simulink library "dab_single_phase_pwm_modulator"  (R2025b)
settings: Solver=VariableStepAuto  StartTime=0.0  StopTime=10.0  RelTol=1e-3
settings Model: Creator=dbagn  LastModifiedBy=ltnbda

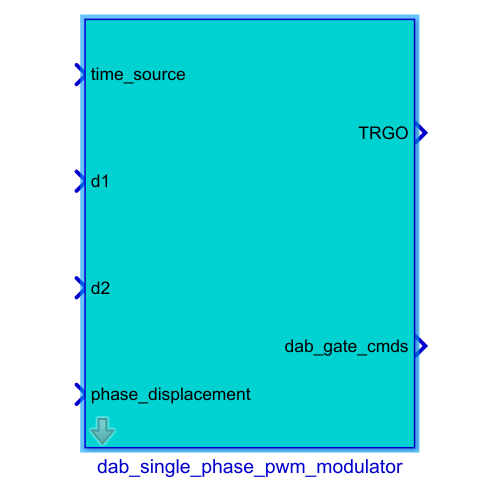
[thumbnail: Simulink's stored preview of the top-level diagram]
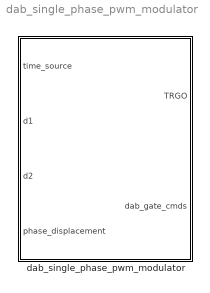
== system dab_single_phase_pwm_modulator ==
  dab_single_phase_pwm_modulator : Subsystem  mask{fPWM_DAB=10000, m_up=1, m_low=0, dead_time_DAB=0, pos_cmd_gate=18, neg_cmd_gate=-3, polarity=-1, tc=1e-6, max_phase_displacement=pi/4, trgo_double_update=0}
      mask prompts: fPWM_DAB "PWM Frequency (Hz)"; m_up "Max Input Modulation Value"; m_low "Min Input Modulation Value"; dead_time_DAB "Dead Time (s)"; pos_cmd_gate "Positive Gate Voltage cmd (V)"; neg_cmd_gate "Negative Gate Voltage cmd (V)"; polarity "Polarity (pu)"; tc "Sampling time"; max_phase_displacement "Max Phase Displacement"; trgo_double_update "TRGO double update"

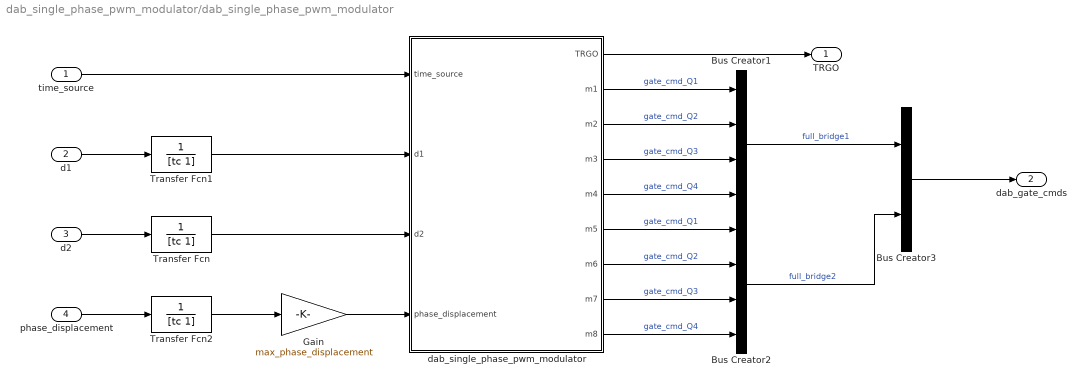
== system dab_single_phase_pwm_modulator/dab_single_phase_pwm_modulator ==
  time_source : Inport
  d1 : Inport  Port=2
  d2 : Inport  Port=3
  phase_displacement : Inport  Port=4
  Bus Creator1 : BusCreator  Inputs=4
  Bus Creator2 : BusCreator  Inputs=4
  Bus Creator3 : BusCreator  Inputs=2
  Gain : Gain  Gain=max_phase_displacement  OutDataTypeStr=double
  Transfer Fcn : TransferFcn  Denominator=[tc 1]
  Transfer Fcn1 : TransferFcn  Denominator=[tc 1]
  Transfer Fcn2 : TransferFcn  Denominator=[tc 1]
  dab_single_phase_pwm_modulator : Subsystem  mask{f=fPWM_DAB, m_up=m_up, m_low=m_low, dead_time=dead_time_DAB, pos_cmd_gate=pos_cmd_gate, neg_cmd_gate=neg_cmd_gate, polarity=polarity, trgo_double_update=trgo_double_update}
      mask prompts: f "Frequency (Hz)"; m_up "Max Input Modulation Value"; m_low "Min Input Modulation Value"; dead_time "Dead Time (s)"; pos_cmd_gate "Positive Gate Voltage (V)"; neg_cmd_gate "Negative Gate Voltage (V)"; polarity "Polarity (pu)"; trgo_double_update "TRGO double update"
  TRGO : Outport
  dab_gate_cmds : Outport  Port=2
  wires:
  d1/1 -> Transfer Fcn1/1
  phase_displacement/1 -> Transfer Fcn2/1
  Gain/1 -> dab_single_phase_pwm_modulator/4(phase_displacement)
  d2/1 -> Transfer Fcn/1
  time_source/1 -> dab_single_phase_pwm_modulator/1(time_source)
  dab_single_phase_pwm_modulator/1(TRGO) -> TRGO/1
  Transfer Fcn1/1 -> dab_single_phase_pwm_modulator/2(d1)
  Transfer Fcn/1 -> dab_single_phase_pwm_modulator/3(d2)
  Transfer Fcn2/1 -> Gain/1
  dab_single_phase_pwm_modulator/2(m1) -> Bus Creator1/1  "gate_cmd_Q1"
  dab_single_phase_pwm_modulator/3(m2) -> Bus Creator1/2  "gate_cmd_Q2"
  dab_single_phase_pwm_modulator/4(m3) -> Bus Creator1/3  "gate_cmd_Q3"
  dab_single_phase_pwm_modulator/5(m4) -> Bus Creator1/4  "gate_cmd_Q4"
  dab_single_phase_pwm_modulator/8(m7) -> Bus Creator2/3  "gate_cmd_Q3"
  dab_single_phase_pwm_modulator/7(m6) -> Bus Creator2/2  "gate_cmd_Q2"
  dab_single_phase_pwm_modulator/6(m5) -> Bus Creator2/1  "gate_cmd_Q1"
  dab_single_phase_pwm_modulator/9(m8) -> Bus Creator2/4  "gate_cmd_Q4"
  Bus Creator3/1 -> dab_gate_cmds/1
  Bus Creator1/1 -> Bus Creator3/1  "full_bridge1"
  Bus Creator2/1 -> Bus Creator3/2  "full_bridge2"

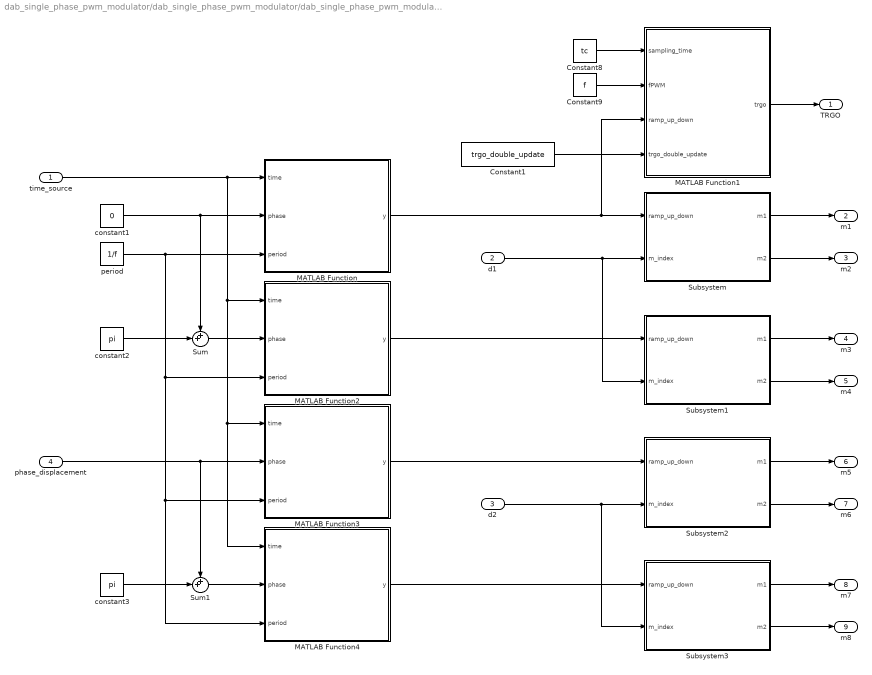
== system dab_single_phase_pwm_modulator/dab_single_phase_pwm_modulator/dab_single_phase_pwm_modulator ==
  time_source : Inport
  d1 : Inport  Port=2
  d2 : Inport  Port=3
  phase_displacement : Inport  Port=4
  Constant1 : Constant  Value=trgo_double_update
  Constant8 : Constant  Value=tc
  Constant9 : Constant  Value=f
  MATLAB Function : MATLAB Function  TreatAsAtomicUnit=on  SystemSampleTime=tc
  MATLAB Function1 : MATLAB Function  TreatAsAtomicUnit=on  SystemSampleTime=tc
  MATLAB Function2 : MATLAB Function  TreatAsAtomicUnit=on  SystemSampleTime=tc
  MATLAB Function3 : MATLAB Function  TreatAsAtomicUnit=on  SystemSampleTime=tc
  MATLAB Function4 : MATLAB Function  TreatAsAtomicUnit=on  SystemSampleTime=tc
  Subsystem : Subsystem
  Subsystem1 : Subsystem
  Subsystem2 : Subsystem
  Subsystem3 : Subsystem
  Sum : Sum  Inputs=++|
  Sum1 : Sum  Inputs=++|
  constant1 : Constant  Value=0
  constant2 : Constant  Value=pi
  "constant3 " : Constant  Value=pi
  period : Constant  Value=1/f
  TRGO : Outport
  m1 : Outport  Port=2
  m2 : Outport  Port=3
  m3 : Outport  Port=4
  m4 : Outport  Port=5
  m5 : Outport  Port=6
  m6 : Outport  Port=7
  m7 : Outport  Port=8
  m8 : Outport  Port=9
  wires:
  MATLAB Function/1(y) -> Subsystem/1(ramp_up_down), MATLAB Function1/3(ramp_up_down)
  Constant8/1 -> MATLAB Function1/1(sampling_time)
  MATLAB Function1/1(trgo) -> TRGO/1
  Constant9/1 -> MATLAB Function1/2(fPWM)
  constant1/1 -> Sum/1, MATLAB Function/2(phase)
  Subsystem/1(m1) -> m1/1
  Subsystem/2(m2) -> m2/1
  Subsystem1/2(m2) -> m4/1
  Subsystem1/1(m1) -> m3/1
  MATLAB Function2/1(y) -> Subsystem1/1(ramp_up_down)
  Sum/1 -> MATLAB Function2/2(phase)
  constant2/1 -> Sum/2
  "constant3 "/1 -> Sum1/2
  Sum1/1 -> MATLAB Function4/2(phase)
  phase_displacement/1 -> MATLAB Function3/2(phase), Sum1/1
  period/1 -> MATLAB Function/3(period), MATLAB Function3/3(period), MATLAB Function4/3(period), MATLAB Function2/3(period)
  time_source/1 -> MATLAB Function/1(time), MATLAB Function3/1(time), MATLAB Function4/1(time), MATLAB Function2/1(time)
  MATLAB Function3/1(y) -> Subsystem2/1(ramp_up_down)
  Subsystem3/1(m1) -> m7/1
  Subsystem3/2(m2) -> m8/1
  Subsystem2/2(m2) -> m6/1
  Subsystem2/1(m1) -> m5/1
  MATLAB Function4/1(y) -> Subsystem3/1(ramp_up_down)
  d1/1 -> Subsystem/2(m_index), Subsystem1/2(m_index)
  d2/1 -> Subsystem3/2(m_index), Subsystem2/2(m_index)
  Constant1/1 -> MATLAB Function1/4(trgo_double_update)

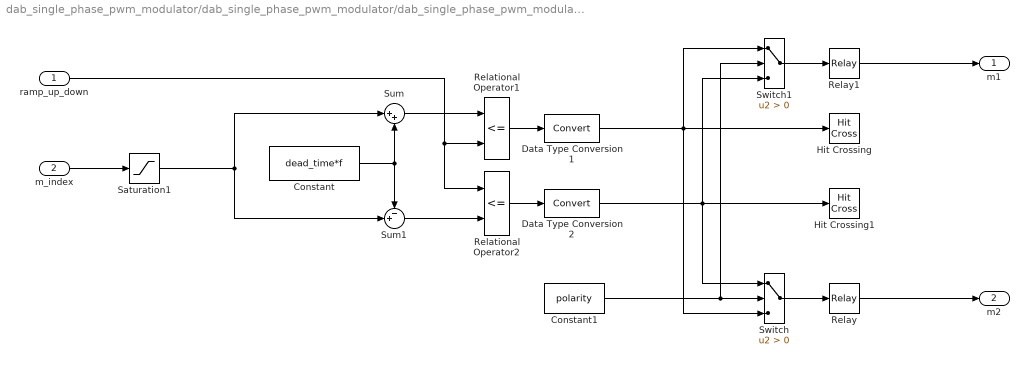
== system dab_single_phase_pwm_modulator/dab_single_phase_pwm_modulator/dab_single_phase_pwm_modulator/Subsystem ==
  ramp_up_down : Inport
  m_index : Inport  Port=2
  Constant : Constant  Value=dead_time*f
  Constant1 : Constant  Value=polarity
  Data Type Conversion1 : DataTypeConversion
  Data Type Conversion2 : DataTypeConversion
  Hit Crossing : HitCross  ShowOutputPort=off
  Hit Crossing1 : HitCross  ShowOutputPort=off
  Relational Operator1 : RelationalOperator  Operator=<=  InputSameDT=off
  Relational Operator2 : RelationalOperator  Operator=<=  InputSameDT=off
  Relay : Relay  OnOutputValue=pos_cmd_gate  OffOutputValue=neg_cmd_gate
  Relay1 : Relay  OnOutputValue=pos_cmd_gate  OffOutputValue=neg_cmd_gate
  Saturation1 : Saturate  UpperLimit=m_up  LowerLimit=m_low
  Sum : Sum  Inputs=|++  SaturateOnIntegerOverflow=on
  Sum1 : Sum  Inputs=-+|  SaturateOnIntegerOverflow=on
  Switch : Switch  Criteria=u2 > Threshold  SaturateOnIntegerOverflow=off  InputSameDT=off
  Switch1 : Switch  Criteria=u2 > Threshold  SaturateOnIntegerOverflow=off  InputSameDT=off
  m1 : Outport
  m2 : Outport  Port=2
  wires:
  Data Type Conversion2/1 -> Switch/1, Switch1/3, Hit Crossing1/1
  Saturation1/1 -> Sum/1, Sum1/2
  Relational Operator2/1 -> Data Type Conversion2/1
  Constant/1 -> Sum/2, Sum1/1
  ramp_up_down/1 -> Relational Operator2/1, Relational Operator1/2
  Switch1/1 -> Relay1/1
  Constant1/1 -> Switch1/2, Switch/2
  m_index/1 -> Saturation1/1
  Relational Operator1/1 -> Data Type Conversion1/1
  Relay/1 -> m2/1
  Relay1/1 -> m1/1
  Data Type Conversion1/1 -> Hit Crossing/1, Switch/3, Switch1/1
  Sum1/1 -> Relational Operator2/2
  Sum/1 -> Relational Operator1/1
  Switch/1 -> Relay/1

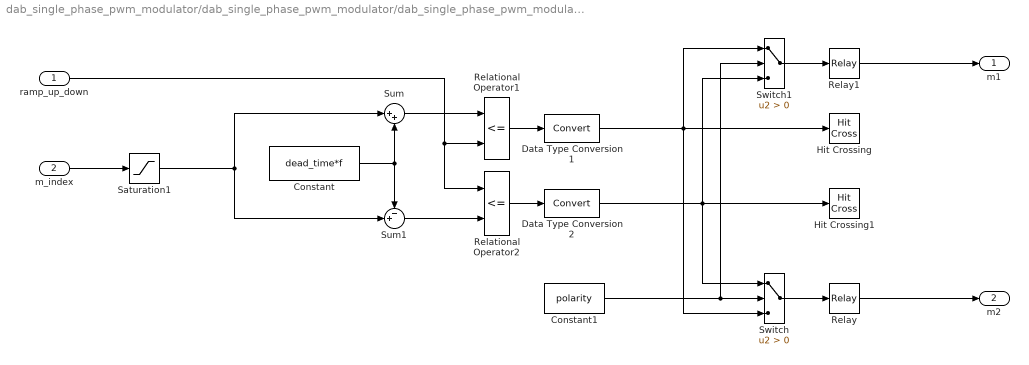
== system dab_single_phase_pwm_modulator/dab_single_phase_pwm_modulator/dab_single_phase_pwm_modulator/Subsystem1 ==
  ramp_up_down : Inport
  m_index : Inport  Port=2
  Constant : Constant  Value=dead_time*f
  Constant1 : Constant  Value=polarity
  Data Type Conversion1 : DataTypeConversion
  Data Type Conversion2 : DataTypeConversion
  Hit Crossing : HitCross  ShowOutputPort=off
  Hit Crossing1 : HitCross  ShowOutputPort=off
  Relational Operator1 : RelationalOperator  Operator=<=  InputSameDT=off
  Relational Operator2 : RelationalOperator  Operator=<=  InputSameDT=off
  Relay : Relay  OnOutputValue=pos_cmd_gate  OffOutputValue=neg_cmd_gate
  Relay1 : Relay  OnOutputValue=pos_cmd_gate  OffOutputValue=neg_cmd_gate
  Saturation1 : Saturate  UpperLimit=m_up  LowerLimit=m_low
  Sum : Sum  Inputs=|++  SaturateOnIntegerOverflow=on
  Sum1 : Sum  Inputs=-+|  SaturateOnIntegerOverflow=on
  Switch : Switch  Criteria=u2 > Threshold  SaturateOnIntegerOverflow=off  InputSameDT=off
  Switch1 : Switch  Criteria=u2 > Threshold  SaturateOnIntegerOverflow=off  InputSameDT=off
  m1 : Outport
  m2 : Outport  Port=2
  wires:
  Switch/1 -> Relay/1
  Sum/1 -> Relational Operator1/1
  Sum1/1 -> Relational Operator2/2
  Data Type Conversion1/1 -> Switch1/1, Switch/3, Hit Crossing/1
  Relay1/1 -> m1/1
  Relay/1 -> m2/1
  Relational Operator1/1 -> Data Type Conversion1/1
  m_index/1 -> Saturation1/1
  Constant1/1 -> Switch/2, Switch1/2
  Switch1/1 -> Relay1/1
  ramp_up_down/1 -> Relational Operator1/2, Relational Operator2/1
  Constant/1 -> Sum1/1, Sum/2
  Relational Operator2/1 -> Data Type Conversion2/1
  Saturation1/1 -> Sum1/2, Sum/1
  Data Type Conversion2/1 -> Hit Crossing1/1, Switch1/3, Switch/1

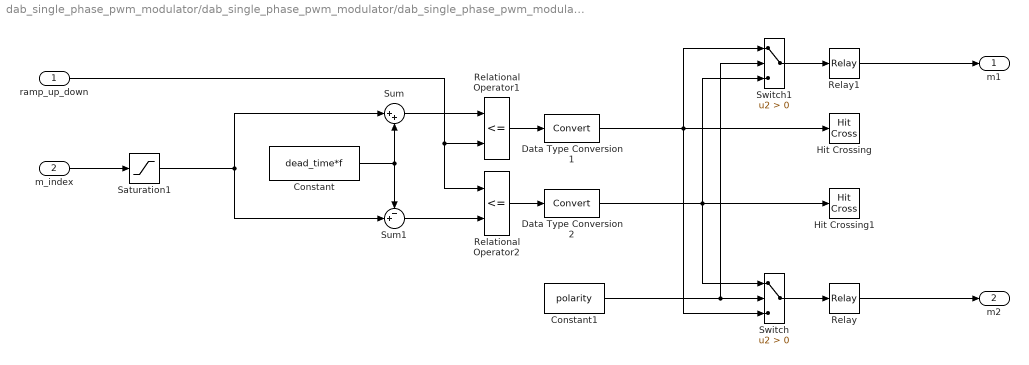
== system dab_single_phase_pwm_modulator/dab_single_phase_pwm_modulator/dab_single_phase_pwm_modulator/Subsystem2 ==
  ramp_up_down : Inport
  m_index : Inport  Port=2
  Constant : Constant  Value=dead_time*f
  Constant1 : Constant  Value=polarity
  Data Type Conversion1 : DataTypeConversion
  Data Type Conversion2 : DataTypeConversion
  Hit Crossing : HitCross  ShowOutputPort=off
  Hit Crossing1 : HitCross  ShowOutputPort=off
  Relational Operator1 : RelationalOperator  Operator=<=  InputSameDT=off
  Relational Operator2 : RelationalOperator  Operator=<=  InputSameDT=off
  Relay : Relay  OnOutputValue=pos_cmd_gate  OffOutputValue=neg_cmd_gate
  Relay1 : Relay  OnOutputValue=pos_cmd_gate  OffOutputValue=neg_cmd_gate
  Saturation1 : Saturate  UpperLimit=m_up  LowerLimit=m_low
  Sum : Sum  Inputs=|++  SaturateOnIntegerOverflow=on
  Sum1 : Sum  Inputs=-+|  SaturateOnIntegerOverflow=on
  Switch : Switch  Criteria=u2 > Threshold  SaturateOnIntegerOverflow=off  InputSameDT=off
  Switch1 : Switch  Criteria=u2 > Threshold  SaturateOnIntegerOverflow=off  InputSameDT=off
  m1 : Outport
  m2 : Outport  Port=2
  wires:
  Data Type Conversion2/1 -> Switch/1, Switch1/3, Hit Crossing1/1
  Saturation1/1 -> Sum/1, Sum1/2
  Relational Operator2/1 -> Data Type Conversion2/1
  Constant/1 -> Sum/2, Sum1/1
  ramp_up_down/1 -> Relational Operator2/1, Relational Operator1/2
  Switch1/1 -> Relay1/1
  Constant1/1 -> Switch1/2, Switch/2
  m_index/1 -> Saturation1/1
  Relational Operator1/1 -> Data Type Conversion1/1
  Relay/1 -> m2/1
  Relay1/1 -> m1/1
  Data Type Conversion1/1 -> Hit Crossing/1, Switch/3, Switch1/1
  Sum1/1 -> Relational Operator2/2
  Sum/1 -> Relational Operator1/1
  Switch/1 -> Relay/1

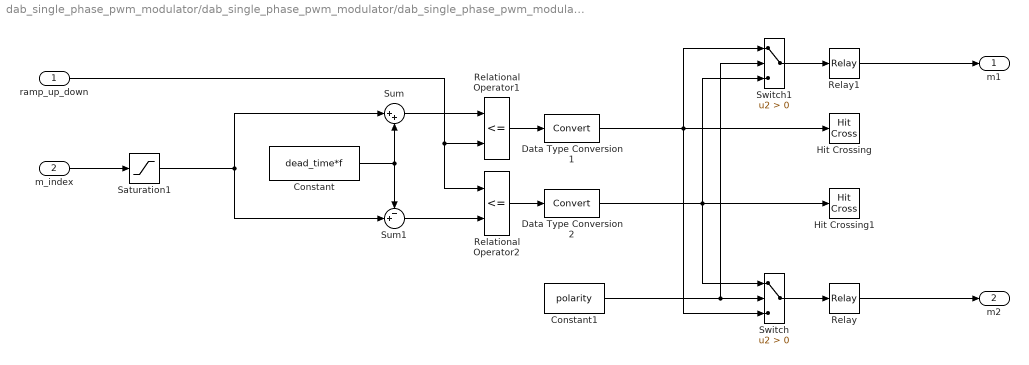
== system dab_single_phase_pwm_modulator/dab_single_phase_pwm_modulator/dab_single_phase_pwm_modulator/Subsystem3 ==
  ramp_up_down : Inport
  m_index : Inport  Port=2
  Constant : Constant  Value=dead_time*f
  Constant1 : Constant  Value=polarity
  Data Type Conversion1 : DataTypeConversion
  Data Type Conversion2 : DataTypeConversion
  Hit Crossing : HitCross  ShowOutputPort=off
  Hit Crossing1 : HitCross  ShowOutputPort=off
  Relational Operator1 : RelationalOperator  Operator=<=  InputSameDT=off
  Relational Operator2 : RelationalOperator  Operator=<=  InputSameDT=off
  Relay : Relay  OnOutputValue=pos_cmd_gate  OffOutputValue=neg_cmd_gate
  Relay1 : Relay  OnOutputValue=pos_cmd_gate  OffOutputValue=neg_cmd_gate
  Saturation1 : Saturate  UpperLimit=m_up  LowerLimit=m_low
  Sum : Sum  Inputs=|++  SaturateOnIntegerOverflow=on
  Sum1 : Sum  Inputs=-+|  SaturateOnIntegerOverflow=on
  Switch : Switch  Criteria=u2 > Threshold  SaturateOnIntegerOverflow=off  InputSameDT=off
  Switch1 : Switch  Criteria=u2 > Threshold  SaturateOnIntegerOverflow=off  InputSameDT=off
  m1 : Outport
  m2 : Outport  Port=2
  wires:
  Switch/1 -> Relay/1
  Sum/1 -> Relational Operator1/1
  Sum1/1 -> Relational Operator2/2
  Data Type Conversion1/1 -> Switch1/1, Switch/3, Hit Crossing/1
  Relay1/1 -> m1/1
  Relay/1 -> m2/1
  Relational Operator1/1 -> Data Type Conversion1/1
  m_index/1 -> Saturation1/1
  Constant1/1 -> Switch/2, Switch1/2
  Switch1/1 -> Relay1/1
  ramp_up_down/1 -> Relational Operator1/2, Relational Operator2/1
  Constant/1 -> Sum1/1, Sum/2
  Relational Operator2/1 -> Data Type Conversion2/1
  Saturation1/1 -> Sum1/2, Sum/1
  Data Type Conversion2/1 -> Hit Crossing1/1, Switch1/3, Switch/1

== matlab function dab_single_phase_pwm_modulator/dab_single_phase_pwm_modulator/MATLAB Function2 ==
  data: time input; y output; phase input; period input
function y = ramp_up_down(time,phase,period)
x = sin(2*pi/period*time - phase -pi/2);
y = asin(x)/pi + 1/2;

== matlab function dab_single_phase_pwm_modulator/dab_single_phase_pwm_modulator/MATLAB Function ==
  data: time input; y output; phase input; period input
function y = ramp_up_down(time,phase,period)
x = sin(2*pi/period*time - phase -pi/2);
y = asin(x)/pi + 1/2;

== matlab function dab_single_phase_pwm_modulator/dab_single_phase_pwm_modulator/MATLAB Function1 ==
  data: sampling_time input; fPWM input; ramp_up_down input; trgo output; trgo_double_update input
function trgo = trgo_gen(sampling_time,fPWM, ramp_up_down, trgo_double_update)

th = fPWM*sampling_time*2;

if trgo_double_update
    if (((ramp_up_down >= 0) && (ramp_up_down <= th)) || ...
            ((ramp_up_down <= 1) && (ramp_up_down >= 1-th)))
        trgo = 1;
    else
        trgo = 0;
    end
else
    if ((ramp_up_down >= 0) && (ramp_up_down <= th))
        trgo = 1;
    else
        trgo = 0;
    end
end

== matlab function dab_single_phase_pwm_modulator/dab_single_phase_pwm_modulator/MATLAB Function3 ==
  data: time input; y output; phase input; period input
function y = ramp_up_down(time,phase,period)
x = sin(2*pi/period*time - phase -pi/2);
y = asin(x)/pi + 1/2;

== matlab function dab_single_phase_pwm_modulator/dab_single_phase_pwm_modulator/MATLAB Function4 ==
  data: time input; y output; phase input; period input
function y = ramp_up_down(time,phase,period)
x = sin(2*pi/period*time - phase -pi/2);
y = asin(x)/pi + 1/2;
